simulink subsystem "q2DCM"  (R2024b)
settings: Solver=VariableStepAuto  StartTime=0.0  StopTime=10.0  RelTol=1e-3
settings Model: Creator=ferru  LastModifiedBy=domac

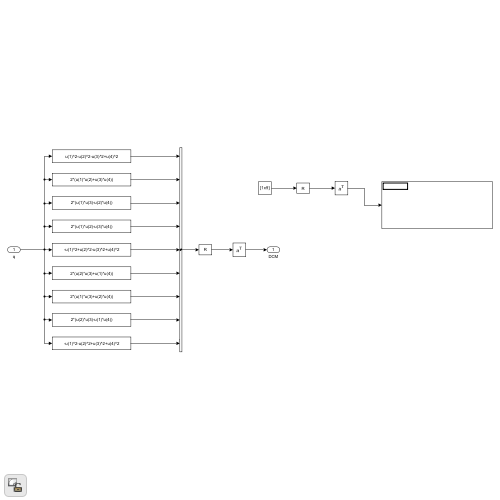
[thumbnail: Simulink's stored preview of the top-level diagram]
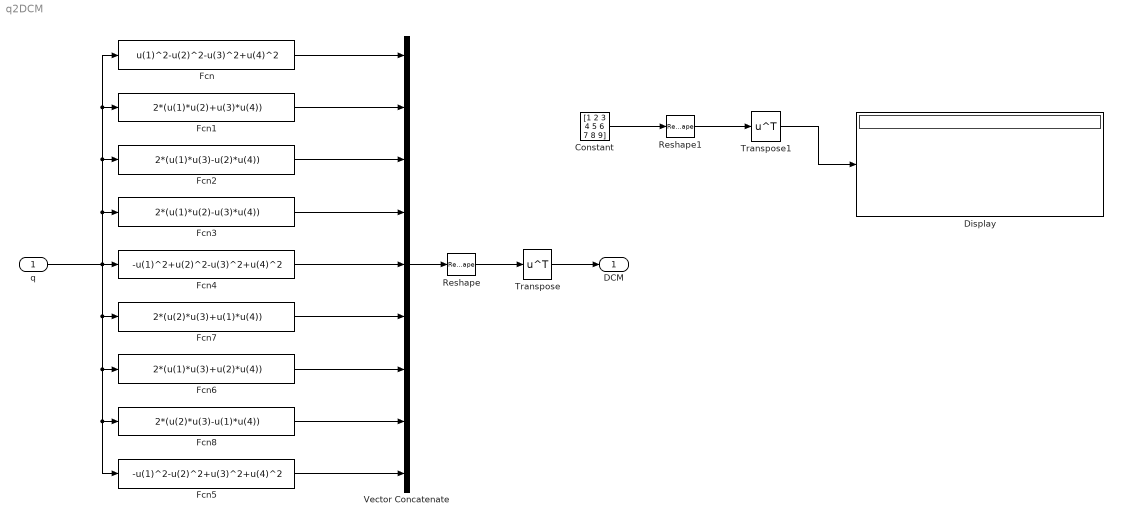
== system q2DCM ==
  q : Inport
  Constant : Constant  Value=[1 2 3 4 5 6 7 8 9]
  Display : Display
  Fcn : Fcn  Expr=u(1)^2-u(2)^2-u(3)^2+u(4)^2
  Fcn1 : Fcn  Expr=2*(u(1)*u(2)+u(3)*u(4))
  Fcn2 : Fcn  Expr=2*(u(1)*u(3)-u(2)*u(4))
  Fcn3 : Fcn  Expr=2*(u(1)*u(2)-u(3)*u(4))
  Fcn4 : Fcn  Expr=-u(1)^2+u(2)^2-u(3)^2+u(4)^2
  Fcn5 : Fcn  Expr=-u(1)^2-u(2)^2+u(3)^2+u(4)^2
  Fcn6 : Fcn  Expr=2*(u(1)*u(3)+u(2)*u(4))
  Fcn7 : Fcn  Expr=2*(u(2)*u(3)+u(1)*u(4))
  Fcn8 : Fcn  Expr=2*(u(2)*u(3)-u(1)*u(4))
  Reshape : Reshape  OutputDimensionality=Customize  OutputDimensions=[3, 3]
  Reshape1 : Reshape  OutputDimensionality=Customize  OutputDimensions=[3, 3]
  Transpose : Math  Operator=transpose
  Transpose1 : Math  Operator=transpose
  Vector Concatenate : Concatenate  NumInputs=9  Mode=Multidimensional array  ConcatenateDimension=2
  DCM : Outport
  wires:
  q/1 -> Fcn3/1, Fcn1/1, Fcn/1, Fcn2/1, Fcn4/1, Fcn8/1, Fcn5/1, Fcn6/1, Fcn7/1
  Fcn/1 -> Vector Concatenate/1
  Fcn1/1 -> Vector Concatenate/2
  Fcn2/1 -> Vector Concatenate/3
  Fcn3/1 -> Vector Concatenate/4
  Fcn4/1 -> Vector Concatenate/5
  Fcn7/1 -> Vector Concatenate/6
  Fcn6/1 -> Vector Concatenate/7
  Fcn8/1 -> Vector Concatenate/8
  Fcn5/1 -> Vector Concatenate/9
  Vector Concatenate/1 -> Reshape/1
  Reshape/1 -> Transpose/1
  Transpose/1 -> DCM/1
  Constant/1 -> Reshape1/1
  Reshape1/1 -> Transpose1/1
  Transpose1/1 -> Display/1
